simulink model "modelo_linear"  (R2025a)
settings: Solver=VariableStepAuto  StartTime=0.0  StopTime=100  RelTol=1e-3
undefined symbols (not defined in the file): A_lat, A_long, B_lat, B_long, C_lat, C_long, D_lat, D_long, Xe, Xe_long
libraries: slpidlib x4
settings Model: Creator=guilh  LastModifiedBy=Kaue

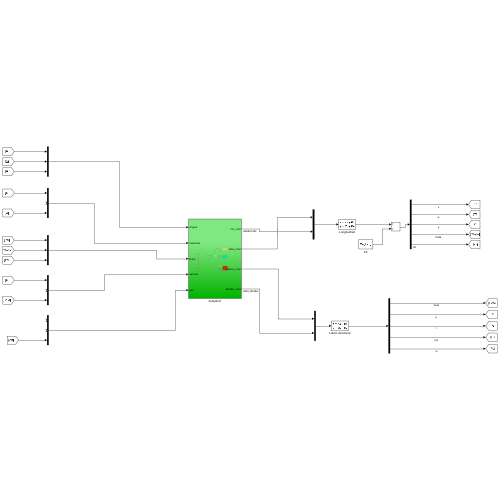
[thumbnail: Simulink's stored preview of the top-level diagram]
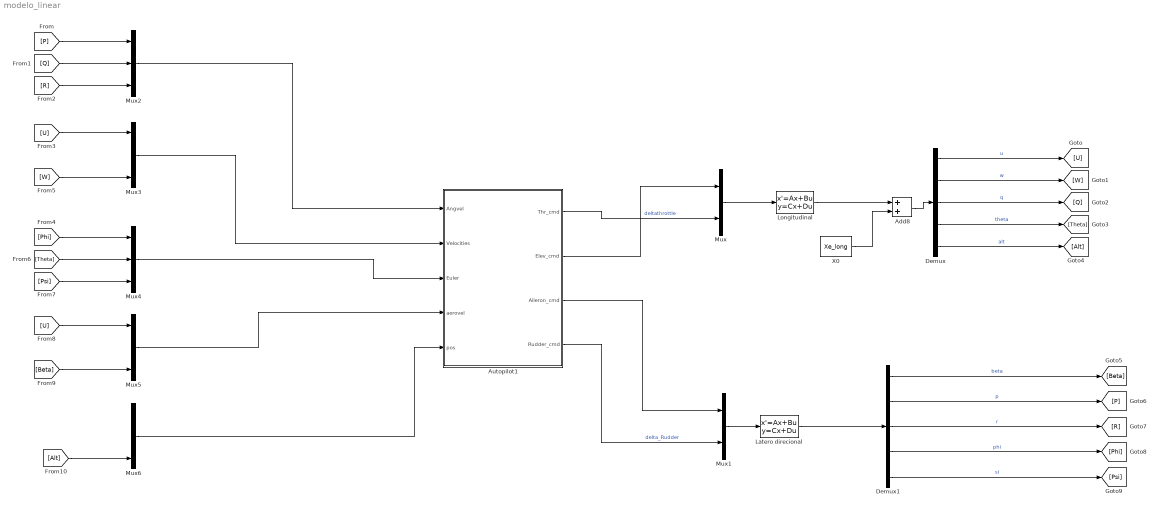
== system modelo_linear ==
  Add8 : Sum
  Autopilot1 : Subsystem
  Demux : Demux  Outputs=5
  Demux1 : Demux  Outputs=5
  Latero direcional : StateSpace  A=A_lat  B=B_lat  C=C_lat  D=D_lat  InitialCondition=0
  Longitudinal : StateSpace  A=A_long  B=B_long  C=C_long  D=D_long  InitialCondition=0
  Mux : Mux  Inputs=2
  Mux1 : Mux  Inputs=2
  Mux{2..6} (5 alike) : Mux  Inputs=3
  X0 : Constant  Value=Xe_long
  wires:
  Mux/1 -> Longitudinal/1
  Mux1/1 -> Latero direcional/1
  Demux/1 -> [U]  "u"
  Demux/2 -> [W]  "w"
  Demux/3 -> [Q]  "q"
  Demux/4 -> [Theta]  "theta"
  Add8/1 -> Demux/1
  Longitudinal/1 -> Add8/1
  X0/1 -> Add8/2
  Latero direcional/1 -> Demux1/1
  Demux1/1 -> [Beta]  "beta"
  Demux1/2 -> [P]  "p"
  Demux1/3 -> [R]  "r"
  Demux1/4 -> [Phi]  "phi"
  Mux2/1 -> Autopilot1/1(Angvel)
  Demux/5 -> [Alt]  "alt"
  Mux3/1 -> Autopilot1/2(Velocities)
  Mux4/1 -> Autopilot1/3(Euler)
  Mux5/1 -> Autopilot1/4(aerovel)
  Mux6/1 -> Autopilot1/5(pos)
  Demux1/5 -> [Psi]  "si"
  [P] -> Mux2/1
  [Q] -> Mux2/2
  [R] -> Mux2/3
  [U] -> Mux3/1
  [W] -> Mux3/3
  [Theta] -> Mux4/2
  [Phi] -> Mux4/1
  [Psi] -> Mux4/3
  [U] -> Mux5/1
  [Beta] -> Mux5/3
  [Alt] -> Mux6/3
  Autopilot1/3(Aileron_cmd) -> Mux1/1
  Autopilot1/4(Rudder_cmd) -> Mux1/2  "delta_Rudder"
  Autopilot1/2(Elev_cmd) -> Mux/1
  Autopilot1/1(Thr_cmd) -> Mux/2  "deltathrottle"

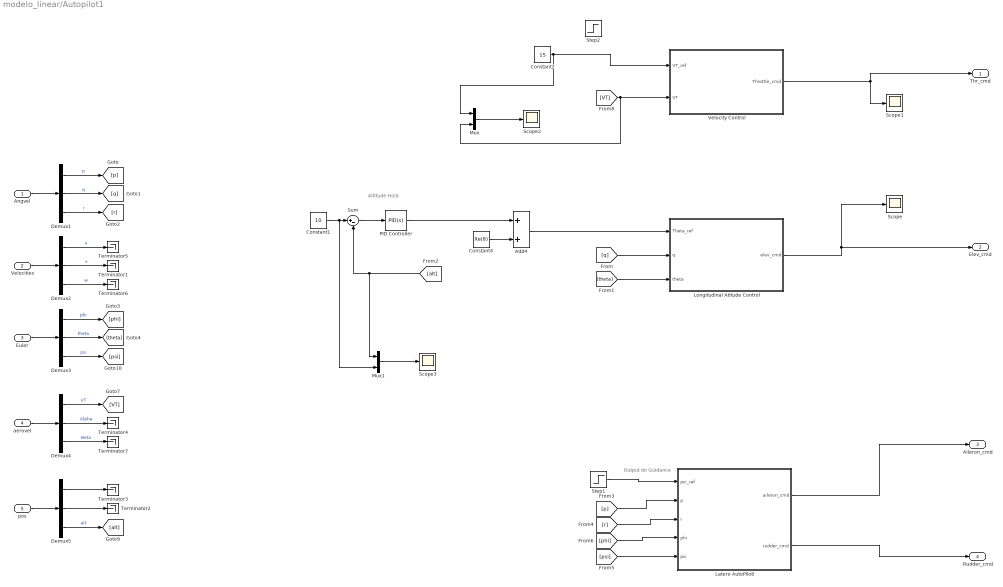
== system modelo_linear/Autopilot1 ==
  note: Altitude Hold
  note: Output do Guidance
  Angvel : Inport
  Velocities : Inport  Port=2
  Euler : Inport  Port=3
  aerovel : Inport  Port=4
  pos : Inport  Port=5
  Add4 : Sum
  Constant1 : Constant  Value=10
  Constant2 : Constant  Value=15
  Constant4 : Constant  Value=Xe(8)
  Demux{1..5} (5 alike) : Demux  Outputs=3
  Latero AutoPilotl : Subsystem
  Longitudinal Atitude Control : Subsystem
  Mux : Mux  Inputs=2
  Mux1 : Mux  Inputs=2
  PID Controller : slpidlib/PID Controller  Controller=PID  Form=Parallel  TimeDomain=Continuous-time  UseExternalTs=off  SampleTime=-1  IntegratorMethod=Forward Euler  FilterMethod=Forward Euler  ControllerParametersSource=internal  P=0.596304245000559  I=0.356254495459697  UseKiTs=off  D=-0.0141697733728916  UseExternalDerivativeSource=off  N=6.17157424867561  UseFilter=on  TunerSelectOption=Transfer Function Based (PID Tuner App)  InitialConditionSource=internal  InitialConditionForIntegrator=0  InitialConditionForFilter=0  DifferentiatorICPrevScaledInput=0  ExternalReset=none  TrackingMode=off  Kt=1  LimitOutput=on  SatLimitsSource=internal  UpperSaturationLimit=0.26  LowerSaturationLimit=-0.17  LinearizeAsGain=on  AntiWindupMode=clamping  Kb=1  LimitIntegrator=off  UpperIntegratorSaturationLimit=inf  LowerIntegratorSaturationLimit=-inf  POutMin=[]  POutMax=[]  IOutMin=[]  IOutMax=[]  DOutMin=[]  DOutMax=[]  NOutMin=[]  NOutMax=[]  SumOutMin=[]  SumOutMax=[]  SaturationOutMin=[]  SaturationOutMax=[]  PParamMin=[]  PParamMax=[]  IParamMin=[]  IParamMax=[]  DParamMin=[]  DParamMax=[]  NParamMin=[]  NParamMax=[]  KbParamMin=[]  KbParamMax=[]  KtParamMin=[]  KtParamMax=[]  KbOutMin=[]  KbOutMax=[]  KtOutMin=[]  KtOutMax=[]  IntegratorOutMin=[]  IntegratorOutMax=[]  FilterOutMin=[]  FilterOutMax=[]  SumI1OutMin=[]  SumI1OutMax=[]  SumI2OutMin=[]  SumI2OutMax=[]  SumI3OutMin=[]  SumI3OutMax=[]  SumI4OutMin=[]  SumI4OutMax=[]  SumDOutMin=[]  SumDOutMax=[]  DifferentiatorOutMin=[]  DifferentiatorOutMax=[]  FilterDiffOutCoefMin=[]  FilterDiffOutCoefMax=[]  ReciprocalOutMin=[]  ReciprocalOutMax=[]  SumDenOutMin=[]  SumDenOutMax=[]  SumNumOutMin=[]  SumNumOutMax=[]  DivideOutMin=[]  DivideOutMax=[]  UdiffTsProdOutMin=[]  UdiffTsProdOutMax=[]  NTsProdOutMin=[]  NTsProdOutMax=[]  UintegralTsProdOutMin=[]  UintegralTsProdOutMax=[]  UngainTsProdOutMin=[]  UngainTsProdOutMax=[]  ClampingZeroOutDataTypeStr=Inherit: Inherit via back propagation  ClampingZeroOutMin=[]  ClampingZeroOutMax=[]  FilterDenConstantOutDataTypeStr=Inherit: Inherit via back propagation  FilterDenConstantOutMin=[]  FilterDenConstantOutMax=[]  PCopyOutDataTypeStr=Inherit: Inherit via back propagation  PCopyOutMin=[]  PCopyOutMax=[]  NCopyOutDataTypeStr=Inherit: Inherit via back propagation  NCopyOutMin=[]  NCopyOutMax=[]  IntegratorContinuousStateAttributes=''  IntegratorStateMustResolveToSignalObject=off  IntegratorRTWStateStorageClass=Auto  FilterContinuousStateAttributes=''  FilterStateMustResolveToSignalObject=off  FilterRTWStateStorageClass=Auto  ParallelPVariant=InternalParameters  IdealPVariant=Disabled  IVariant=InternalParameters  DVariant=InternalParameters  IntegratorVariant=Continuous  SatVariant=Enabled  AWVariant=ContClampingParallel  PCopyVariant=Disabled  TRVariant=Disabled  FdbkBlocksVariant=Forward  IdealPFdbkVariant=Disabled  SatFdbkVariant=Disabled  DerivativeFilterVariant=ContFilter  NVariant=InternalParameters  NCopyVariant=Disabled  FilterICVariant=InternalICsFilter  IntegratorICVariant=InternalICs  ExternalResetVariant=Disabled  TRSumVariant=Passthrough  SumFdbkVariant=Disabled  SumVariant=Sum_PID  TsampFilterVariant=InternalTs  TsampNgainVariant=Passthrough  TsampIntegralVariant=Disabled_SignalSpec  ExternalSaturationOutDataTypeStr=Inherit: Same as second input  DerivativeSourceVariant=ErrorSignal  PreIntVariant=InternalPreInt
  Scope{,1..3} (4 alike) : Scope
      Scope settings: ActiveDisplayYMinimum=-0.35368  ActiveDisplayYMaximum=2.71315
      Scope1 settings: ActiveDisplayYMinimum=-175.42515203895346  ActiveDisplayYMaximum=154.54522885010272  DataLoggingVariableName=ScopeData2
      Scope2 settings: ActiveDisplayYMinimum=5.9588664236707132  ActiveDisplayYMaximum=17.571708011531506  DataLoggingVariableName=ScopeData4
      Scope3 settings: ActiveDisplayYMinimum=-87.496956287029832  ActiveDisplayYMaximum=10.567340507352135  DataLoggingVariableName=ScopeData7
  Step1 : Step  Time=5  After=deg2rad(50)  SampleTime=0
  Step2 : Step  Time=5  Before=15  After=18  SampleTime=0.01
  Sum : Sum  Inputs=|+-
  Terminator{1..7} (7 alike) : Terminator
  Velocity Control : Subsystem
  Thr_cmd : Outport
  Elev_cmd : Outport  Port=2
  Aileron_cmd : Outport  Port=3
  Rudder_cmd : Outport  Port=4
  wires:
  Angvel/1 -> Demux1/1
  Velocities/1 -> Demux2/1
  Demux1/1 -> [p]  "p"
  Demux1/2 -> [q]  "q"
  Demux1/3 -> [r]  "r"
  Euler/1 -> Demux3/1
  Demux3/3 -> [psi]  "psi"
  Demux3/1 -> [phi]  "phi"
  Demux3/2 -> [theta]  "theta"
  Demux2/3 -> Terminator6/1  "w"
  Demux2/1 -> Terminator5/1  "u"
  Demux2/2 -> Terminator1/1  "v"
  [theta] -> Longitudinal Atitude Control/3(theta)
  aerovel/1 -> Demux4/1
  Demux4/1 -> [VT]  "VT"
  Demux4/2 -> Terminator4/1  "Alpha"
  Demux4/3 -> Terminator7/1  "Beta"
  Velocity Control/1(Throttle_cmd) -> Thr_cmd/1, Scope1/1
  Latero AutoPilotl/1(aileron_cmd) -> Aileron_cmd/1
  Latero AutoPilotl/2(rudder_cmd) -> Rudder_cmd/1
  [q] -> Longitudinal Atitude Control/2(q)
  Longitudinal Atitude Control/1(elev_cmd) -> Elev_cmd/1, Scope/1
  [VT] -> Mux/2, Velocity Control/2(VT)
  pos/1 -> Demux5/1
  Demux5/3 -> [alt]  "alt"
  Demux5/2 -> Terminator2/1
  Demux5/1 -> Terminator3/1
  [alt] -> Mux1/1, Sum/2
  Sum/1 -> PID Controller/1
  [p] -> Latero AutoPilotl/2(p)
  [r] -> Latero AutoPilotl/3(r)
  [psi] -> Latero AutoPilotl/5(psi)
  [phi] -> Latero AutoPilotl/4(phi)
  Constant4/1 -> Add4/2
  Step1/1 -> Latero AutoPilotl/1(psi_ref)
  PID Controller/1 -> Add4/1
  Constant1/1 -> Mux1/2, Sum/1
  Mux/1 -> Scope2/1
  Add4/1 -> Longitudinal Atitude Control/1(Theta_ref)
  Mux1/1 -> Scope3/1
  Constant2/1 -> Mux/1, Velocity Control/1(VT_ref)

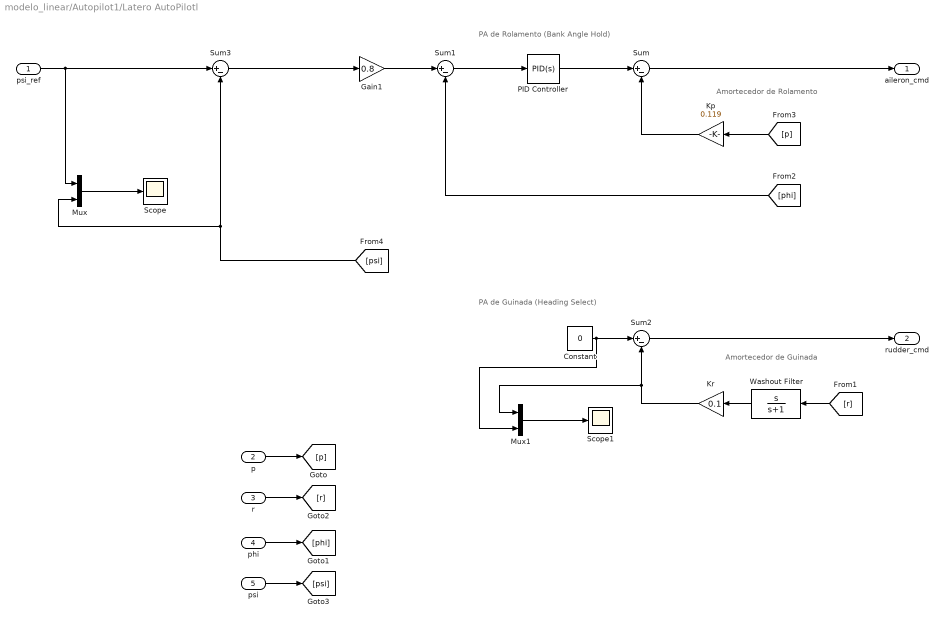
== system modelo_linear/Autopilot1/Latero AutoPilotl ==
  note: PA de Rolamento (Bank Angle Hold)
  note: Amortecedor de Rolamento
  note: Amortecedor de Guinada
  note: PA de Guinada (Heading Select)
  psi_ref : Inport
  p : Inport  Port=2
  r : Inport  Port=3
  phi : Inport  Port=4
  psi : Inport  Port=5
  Constant : Constant  Value=0
  Gain1 : Gain  Gain=0.8
  Kp : Gain  Gain=0.119
  Kr : Gain  Gain=0.1
  Mux : Mux  Inputs=2
  Mux1 : Mux  Inputs=2
  PID Controller : slpidlib/PID Controller  Controller=PID  Form=Parallel  TimeDomain=Continuous-time  UseExternalTs=off  SampleTime=-1  IntegratorMethod=Forward Euler  FilterMethod=Forward Euler  ControllerParametersSource=internal  P=26.7874562402529  I=13.1675046432808  UseKiTs=off  D=-0.0875715773472267  UseExternalDerivativeSource=off  N=305.892129064194  UseFilter=on  TunerSelectOption=Transfer Function Based (PID Tuner App)  InitialConditionSource=internal  InitialConditionForIntegrator=0  InitialConditionForFilter=0  DifferentiatorICPrevScaledInput=0  ExternalReset=none  TrackingMode=off  Kt=1  LimitOutput=off  SatLimitsSource=internal  UpperSaturationLimit=inf  LowerSaturationLimit=-inf  LinearizeAsGain=on  AntiWindupMode=none  Kb=1  LimitIntegrator=off  UpperIntegratorSaturationLimit=inf  LowerIntegratorSaturationLimit=-inf  POutMin=[]  POutMax=[]  IOutMin=[]  IOutMax=[]  DOutMin=[]  DOutMax=[]  NOutMin=[]  NOutMax=[]  SumOutMin=[]  SumOutMax=[]  SaturationOutMin=[]  SaturationOutMax=[]  PParamMin=[]  PParamMax=[]  IParamMin=[]  IParamMax=[]  DParamMin=[]  DParamMax=[]  NParamMin=[]  NParamMax=[]  KbParamMin=[]  KbParamMax=[]  KtParamMin=[]  KtParamMax=[]  KbOutMin=[]  KbOutMax=[]  KtOutMin=[]  KtOutMax=[]  IntegratorOutMin=[]  IntegratorOutMax=[]  FilterOutMin=[]  FilterOutMax=[]  SumI1OutMin=[]  SumI1OutMax=[]  SumI2OutMin=[]  SumI2OutMax=[]  SumI3OutMin=[]  SumI3OutMax=[]  SumI4OutMin=[]  SumI4OutMax=[]  SumDOutMin=[]  SumDOutMax=[]  DifferentiatorOutMin=[]  DifferentiatorOutMax=[]  FilterDiffOutCoefMin=[]  FilterDiffOutCoefMax=[]  ReciprocalOutMin=[]  ReciprocalOutMax=[]  SumDenOutMin=[]  SumDenOutMax=[]  SumNumOutMin=[]  SumNumOutMax=[]  DivideOutMin=[]  DivideOutMax=[]  UdiffTsProdOutMin=[]  UdiffTsProdOutMax=[]  NTsProdOutMin=[]  NTsProdOutMax=[]  UintegralTsProdOutMin=[]  UintegralTsProdOutMax=[]  UngainTsProdOutMin=[]  UngainTsProdOutMax=[]  ClampingZeroOutDataTypeStr=Inherit: Inherit via back propagation  ClampingZeroOutMin=[]  ClampingZeroOutMax=[]  FilterDenConstantOutDataTypeStr=Inherit: Inherit via back propagation  FilterDenConstantOutMin=[]  FilterDenConstantOutMax=[]  PCopyOutDataTypeStr=Inherit: Inherit via back propagation  PCopyOutMin=[]  PCopyOutMax=[]  NCopyOutDataTypeStr=Inherit: Inherit via back propagation  NCopyOutMin=[]  NCopyOutMax=[]  IntegratorContinuousStateAttributes=''  IntegratorStateMustResolveToSignalObject=off  IntegratorRTWStateStorageClass=Auto  FilterContinuousStateAttributes=''  FilterStateMustResolveToSignalObject=off  FilterRTWStateStorageClass=Auto  ParallelPVariant=InternalParameters  IdealPVariant=Disabled  IVariant=InternalParameters  DVariant=InternalParameters  IntegratorVariant=Continuous  SatVariant=Disabled  AWVariant=Passthrough  PCopyVariant=Disabled  TRVariant=Disabled  FdbkBlocksVariant=Forward  IdealPFdbkVariant=Disabled  SatFdbkVariant=Disabled  DerivativeFilterVariant=ContFilter  NVariant=InternalParameters  NCopyVariant=Disabled  FilterICVariant=InternalICsFilter  IntegratorICVariant=InternalICs  ExternalResetVariant=Disabled  TRSumVariant=Passthrough  SumFdbkVariant=Disabled  SumVariant=Sum_PID  TsampFilterVariant=InternalTs  TsampNgainVariant=Passthrough  TsampIntegralVariant=Disabled_SignalSpec  ExternalSaturationOutDataTypeStr=Inherit: Same as second input  DerivativeSourceVariant=ErrorSignal  PreIntVariant=InternalPreInt
  Scope : Scope
      settings: ActiveDisplayYMinimum=-1  ActiveDisplayYMaximum=1  DataLoggingVariableName=ScopeData5
  Scope1 : Scope
      settings: ActiveDisplayYMinimum=-0.31235  ActiveDisplayYMaximum=0.29284  DataLoggingVariableName=ScopeData2
  Sum{,1..3} (4 alike) : Sum  Inputs=|+-
  Washout Filter : TransferFcn  Numerator=[1 0]  Denominator=[1 1]
  aileron_cmd : Outport
  rudder_cmd : Outport  Port=2
  wires:
  Sum1/1 -> PID Controller/1
  Sum/1 -> aileron_cmd/1
  [p] -> Kp/1
  [phi] -> Sum1/2
  Kp/1 -> Sum/2
  PID Controller/1 -> Sum/1
  p/1 -> [p]
  [r] -> Washout Filter/1
  Kr/1 -> Mux1/1, Sum2/2
  r/1 -> [r]
  Washout Filter/1 -> Kr/1
  phi/1 -> [phi]
  psi/1 -> [psi]
  Sum3/1 -> Gain1/1
  [psi] -> Sum3/2, Mux/2
  psi_ref/1 -> Mux/1, Sum3/1
  Sum2/1 -> rudder_cmd/1
  Constant/1 -> Mux1/2, Sum2/1
  Gain1/1 -> Sum1/1
  Mux/1 -> Scope/1
  Mux1/1 -> Scope1/1

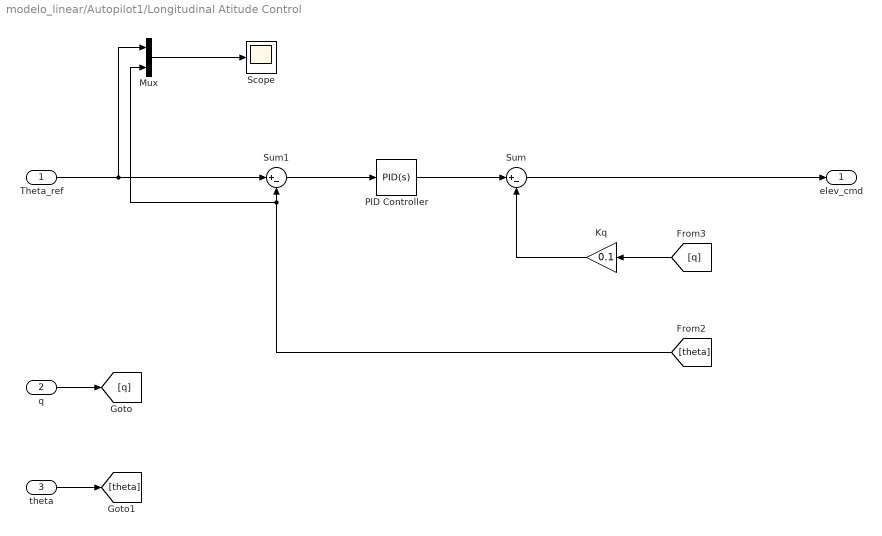
== system modelo_linear/Autopilot1/Longitudinal Atitude Control ==
  Theta_ref : Inport
  q : Inport  Port=2
  theta : Inport  Port=3
  Kq : Gain  Gain=0.1
  Mux : Mux  Inputs=2
  PID Controller : slpidlib/PID Controller  Controller=PID  Form=Parallel  TimeDomain=Continuous-time  UseExternalTs=off  SampleTime=-1  IntegratorMethod=Forward Euler  FilterMethod=Forward Euler  ControllerParametersSource=internal  P=20.3142831421082  I=22.5973845921282  UseKiTs=off  D=1.76724278063426  UseExternalDerivativeSource=off  N=1159.39165466191  UseFilter=on  TunerSelectOption=Transfer Function Based (PID Tuner App)  InitialConditionSource=internal  InitialConditionForIntegrator=0  InitialConditionForFilter=0  DifferentiatorICPrevScaledInput=0  ExternalReset=none  TrackingMode=off  Kt=1  LimitOutput=off  SatLimitsSource=internal  UpperSaturationLimit=inf  LowerSaturationLimit=-inf  LinearizeAsGain=on  AntiWindupMode=none  Kb=1  LimitIntegrator=off  UpperIntegratorSaturationLimit=inf  LowerIntegratorSaturationLimit=-inf  POutMin=[]  POutMax=[]  IOutMin=[]  IOutMax=[]  DOutMin=[]  DOutMax=[]  NOutMin=[]  NOutMax=[]  SumOutMin=[]  SumOutMax=[]  SaturationOutMin=[]  SaturationOutMax=[]  PParamMin=[]  PParamMax=[]  IParamMin=[]  IParamMax=[]  DParamMin=[]  DParamMax=[]  NParamMin=[]  NParamMax=[]  KbParamMin=[]  KbParamMax=[]  KtParamMin=[]  KtParamMax=[]  KbOutMin=[]  KbOutMax=[]  KtOutMin=[]  KtOutMax=[]  IntegratorOutMin=[]  IntegratorOutMax=[]  FilterOutMin=[]  FilterOutMax=[]  SumI1OutMin=[]  SumI1OutMax=[]  SumI2OutMin=[]  SumI2OutMax=[]  SumI3OutMin=[]  SumI3OutMax=[]  SumI4OutMin=[]  SumI4OutMax=[]  SumDOutMin=[]  SumDOutMax=[]  DifferentiatorOutMin=[]  DifferentiatorOutMax=[]  FilterDiffOutCoefMin=[]  FilterDiffOutCoefMax=[]  ReciprocalOutMin=[]  ReciprocalOutMax=[]  SumDenOutMin=[]  SumDenOutMax=[]  SumNumOutMin=[]  SumNumOutMax=[]  DivideOutMin=[]  DivideOutMax=[]  UdiffTsProdOutMin=[]  UdiffTsProdOutMax=[]  NTsProdOutMin=[]  NTsProdOutMax=[]  UintegralTsProdOutMin=[]  UintegralTsProdOutMax=[]  UngainTsProdOutMin=[]  UngainTsProdOutMax=[]  ClampingZeroOutDataTypeStr=Inherit: Inherit via back propagation  ClampingZeroOutMin=[]  ClampingZeroOutMax=[]  FilterDenConstantOutDataTypeStr=Inherit: Inherit via back propagation  FilterDenConstantOutMin=[]  FilterDenConstantOutMax=[]  PCopyOutDataTypeStr=Inherit: Inherit via back propagation  PCopyOutMin=[]  PCopyOutMax=[]  NCopyOutDataTypeStr=Inherit: Inherit via back propagation  NCopyOutMin=[]  NCopyOutMax=[]  IntegratorContinuousStateAttributes=''  IntegratorStateMustResolveToSignalObject=off  IntegratorRTWStateStorageClass=Auto  FilterContinuousStateAttributes=''  FilterStateMustResolveToSignalObject=off  FilterRTWStateStorageClass=Auto  ParallelPVariant=InternalParameters  IdealPVariant=Disabled  IVariant=InternalParameters  DVariant=InternalParameters  IntegratorVariant=Continuous  SatVariant=Disabled  AWVariant=Passthrough  PCopyVariant=Disabled  TRVariant=Disabled  FdbkBlocksVariant=Forward  IdealPFdbkVariant=Disabled  SatFdbkVariant=Disabled  DerivativeFilterVariant=ContFilter  NVariant=InternalParameters  NCopyVariant=Disabled  FilterICVariant=InternalICsFilter  IntegratorICVariant=InternalICs  ExternalResetVariant=Disabled  TRSumVariant=Passthrough  SumFdbkVariant=Disabled  SumVariant=Sum_PID  TsampFilterVariant=InternalTs  TsampNgainVariant=Passthrough  TsampIntegralVariant=Disabled_SignalSpec  ExternalSaturationOutDataTypeStr=Inherit: Same as second input  DerivativeSourceVariant=ErrorSignal  PreIntVariant=InternalPreInt
  Scope : Scope
      settings: ActiveDisplayYMinimum=-0.5  ActiveDisplayYMaximum=0.49279  DataLoggingVariableName=ScopeData3
  Sum : Sum  Inputs=|+-
  Sum1 : Sum  Inputs=|+-
  elev_cmd : Outport
  wires:
  Sum1/1 -> PID Controller/1
  Sum/1 -> elev_cmd/1
  [q] -> Kq/1
  [theta] -> Mux/2, Sum1/2
  Kq/1 -> Sum/2
  theta/1 -> [theta]
  q/1 -> [q]
  Theta_ref/1 -> Sum1/1, Mux/1
  Mux/1 -> Scope/1
  PID Controller/1 -> Sum/1

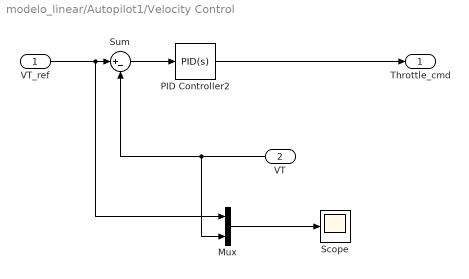
== system modelo_linear/Autopilot1/Velocity Control ==
  VT_ref : Inport
  VT : Inport  Port=2
  Mux : Mux  Inputs=2
  PID Controller2 : slpidlib/PID Controller  Controller=PID  Form=Parallel  TimeDomain=Continuous-time  UseExternalTs=off  SampleTime=-1  IntegratorMethod=Forward Euler  FilterMethod=Forward Euler  ControllerParametersSource=internal  P=-0.0786752433250596  I=-0.0651689570386166  UseKiTs=off  D=-0.0151687829718727  UseExternalDerivativeSource=off  N=77.0155336495376  UseFilter=on  TunerSelectOption=Transfer Function Based (PID Tuner App)  InitialConditionSource=internal  InitialConditionForIntegrator=0  InitialConditionForFilter=0  DifferentiatorICPrevScaledInput=0  ExternalReset=none  TrackingMode=off  Kt=1  LimitOutput=off  SatLimitsSource=internal  UpperSaturationLimit=inf  LowerSaturationLimit=-inf  LinearizeAsGain=on  AntiWindupMode=none  Kb=1  LimitIntegrator=off  UpperIntegratorSaturationLimit=inf  LowerIntegratorSaturationLimit=-inf  POutMin=[]  POutMax=[]  IOutMin=[]  IOutMax=[]  DOutMin=[]  DOutMax=[]  NOutMin=[]  NOutMax=[]  SumOutMin=[]  SumOutMax=[]  SaturationOutMin=[]  SaturationOutMax=[]  PParamMin=[]  PParamMax=[]  IParamMin=[]  IParamMax=[]  DParamMin=[]  DParamMax=[]  NParamMin=[]  NParamMax=[]  KbParamMin=[]  KbParamMax=[]  KtParamMin=[]  KtParamMax=[]  KbOutMin=[]  KbOutMax=[]  KtOutMin=[]  KtOutMax=[]  IntegratorOutMin=[]  IntegratorOutMax=[]  FilterOutMin=[]  FilterOutMax=[]  SumI1OutMin=[]  SumI1OutMax=[]  SumI2OutMin=[]  SumI2OutMax=[]  SumI3OutMin=[]  SumI3OutMax=[]  SumI4OutMin=[]  SumI4OutMax=[]  SumDOutMin=[]  SumDOutMax=[]  DifferentiatorOutMin=[]  DifferentiatorOutMax=[]  FilterDiffOutCoefMin=[]  FilterDiffOutCoefMax=[]  ReciprocalOutMin=[]  ReciprocalOutMax=[]  SumDenOutMin=[]  SumDenOutMax=[]  SumNumOutMin=[]  SumNumOutMax=[]  DivideOutMin=[]  DivideOutMax=[]  UdiffTsProdOutMin=[]  UdiffTsProdOutMax=[]  NTsProdOutMin=[]  NTsProdOutMax=[]  UintegralTsProdOutMin=[]  UintegralTsProdOutMax=[]  UngainTsProdOutMin=[]  UngainTsProdOutMax=[]  ClampingZeroOutDataTypeStr=Inherit: Inherit via back propagation  ClampingZeroOutMin=[]  ClampingZeroOutMax=[]  FilterDenConstantOutDataTypeStr=Inherit: Inherit via back propagation  FilterDenConstantOutMin=[]  FilterDenConstantOutMax=[]  PCopyOutDataTypeStr=Inherit: Inherit via back propagation  PCopyOutMin=[]  PCopyOutMax=[]  NCopyOutDataTypeStr=Inherit: Inherit via back propagation  NCopyOutMin=[]  NCopyOutMax=[]  IntegratorContinuousStateAttributes=''  IntegratorStateMustResolveToSignalObject=off  IntegratorRTWStateStorageClass=Auto  FilterContinuousStateAttributes=''  FilterStateMustResolveToSignalObject=off  FilterRTWStateStorageClass=Auto  ParallelPVariant=InternalParameters  IdealPVariant=Disabled  IVariant=InternalParameters  DVariant=InternalParameters  IntegratorVariant=Continuous  SatVariant=Disabled  AWVariant=Passthrough  PCopyVariant=Disabled  TRVariant=Disabled  FdbkBlocksVariant=Forward  IdealPFdbkVariant=Disabled  SatFdbkVariant=Disabled  DerivativeFilterVariant=ContFilter  NVariant=InternalParameters  NCopyVariant=Disabled  FilterICVariant=InternalICsFilter  IntegratorICVariant=InternalICs  ExternalResetVariant=Disabled  TRSumVariant=Passthrough  SumFdbkVariant=Disabled  SumVariant=Sum_PID  TsampFilterVariant=InternalTs  TsampNgainVariant=Passthrough  TsampIntegralVariant=Disabled_SignalSpec  ExternalSaturationOutDataTypeStr=Inherit: Same as second input  DerivativeSourceVariant=ErrorSignal  PreIntVariant=InternalPreInt
  Scope : Scope
      settings: ActiveDisplayYMinimum=14.2491  ActiveDisplayYMaximum=18.84796
  Sum : Sum  Inputs=|+-
  Throttle_cmd : Outport
  wires:
  VT/1 -> Mux/2, Sum/2
  VT_ref/1 -> Mux/1, Sum/1
  Mux/1 -> Scope/1
  PID Controller2/1 -> Throttle_cmd/1
  Sum/1 -> PID Controller2/1
